simulink model "SDOF_v1"  (R2026a)
settings: Solver=VariableStepAuto  StopTime=200
InitFcn:
  | model_path = fileparts(get_param(bdroot, 'FileName'));
  | parent_path = fileparts(model_path);
  | run(fullfile(parent_path, 'scripts', 'InitFcn.m'));
undefined symbols (not defined in the file): data, envP
libraries: simulink x2
settings Model: Creator=awint  LastModifiedBy=benjaminbrobst

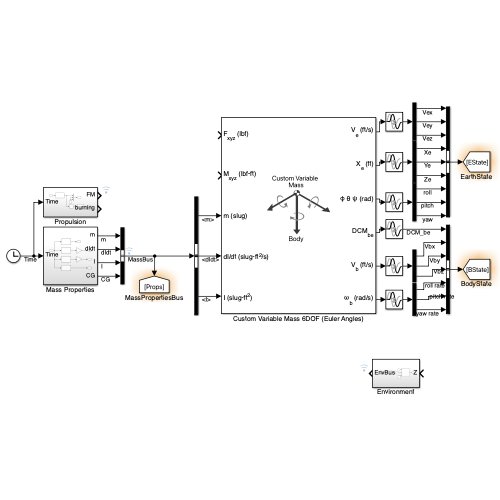
[thumbnail: Simulink's stored preview of the top-level diagram]
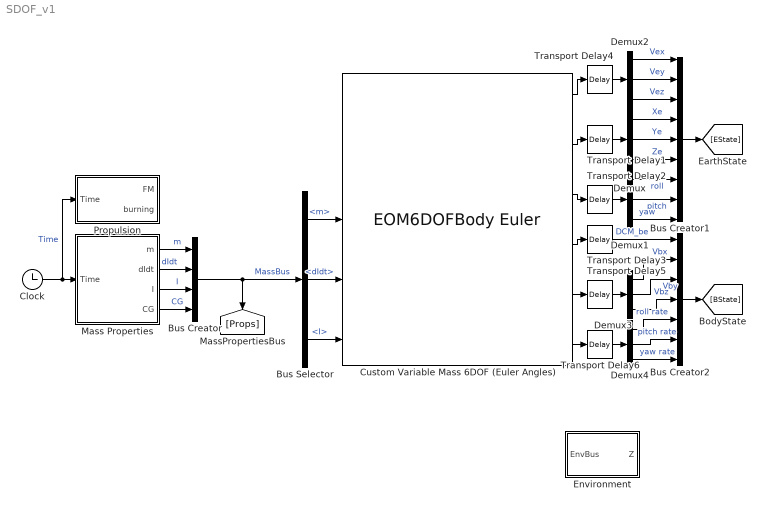
== system SDOF_v1 ==
  Bus Creator : BusCreator  Inputs=4
  Bus Creator1 : BusCreator  Inputs=9
  Bus Creator2 : BusCreator  Inputs=7
  Bus Selector : BusSelector  OutputSignals=m,dIdt,I
  Clock : Clock
  Custom Variable Mass 6DOF (Euler Angles) : EOM6DOFBodyEuler  units=English (velocity in ft/s)  mtype=Custom Variable
  Demux{,1..4} (5 alike) : Demux  Outputs=3
  Environment : Subsystem
  Mass Properties : Subsystem
  Propulsion : Subsystem
  Transport Delay{1..6} (6 alike) : TransportDelay  DelayTime=0.001
  wires:
  Clock/1 -> Propulsion/1(Time), Mass Properties/1(Time)  "Time"
  Custom Variable Mass 6DOF (Euler Angles)/1 -> Transport Delay4/1
  Custom Variable Mass 6DOF (Euler Angles)/2 -> Transport Delay1/1
  Custom Variable Mass 6DOF (Euler Angles)/3 -> Transport Delay2/1
  Custom Variable Mass 6DOF (Euler Angles)/4 -> Transport Delay3/1
  Custom Variable Mass 6DOF (Euler Angles)/5 -> Transport Delay5/1
  Custom Variable Mass 6DOF (Euler Angles)/6 -> Transport Delay6/1
  Mass Properties/4(CG) -> Bus Creator/4  "CG"
  Mass Properties/3(I) -> Bus Creator/3  "I"
  Mass Properties/2(dIdt) -> Bus Creator/2  "dIdt"
  Mass Properties/1(m) -> Bus Creator/1  "m"
  Bus Creator/1 -> Bus Selector/1, [Props]  "MassBus"
  Bus Selector/1 -> Custom Variable Mass 6DOF (Euler Angles)/3  "<m>"
  Bus Selector/2 -> Custom Variable Mass 6DOF (Euler Angles)/4  "<dIdt>"
  Bus Selector/3 -> Custom Variable Mass 6DOF (Euler Angles)/5  "<I>"
  Transport Delay4/1 -> Demux2/1
  Transport Delay1/1 -> Demux/1
  Transport Delay2/1 -> Demux1/1
  Transport Delay5/1 -> Demux3/1
  Transport Delay6/1 -> Demux4/1
  Demux2/1 -> Bus Creator1/1  "Vex"
  Demux2/2 -> Bus Creator1/2  "Vey"
  Demux2/3 -> Bus Creator1/3  "Vez"
  Demux/1 -> Bus Creator1/4  "Xe"
  Demux/2 -> Bus Creator1/5  "Ye"
  Demux/3 -> Bus Creator1/6  "Ze"
  Demux1/1 -> Bus Creator1/7  "roll"
  Demux1/2 -> Bus Creator1/8  "pitch"
  Demux1/3 -> Bus Creator1/9  "yaw"
  Demux4/3 -> Bus Creator2/7  "yaw rate"
  Demux4/2 -> Bus Creator2/6  "pitch rate"
  Demux4/1 -> Bus Creator2/5  "roll rate"
  Demux3/3 -> Bus Creator2/4  "Vbz"
  Demux3/2 -> Bus Creator2/3  "Vby"
  Demux3/1 -> Bus Creator2/2  "Vbx"
  Transport Delay3/1 -> Bus Creator2/1  "DCM_be"
  Bus Creator1/1 -> [EState]
  Bus Creator2/1 -> [BState]

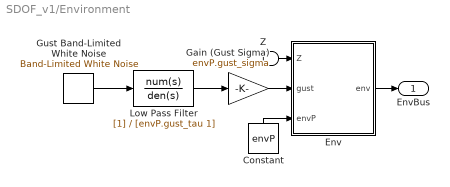
== system SDOF_v1/Environment ==
  Z : Inport
  Constant : Constant  Value=envP  OutDataTypeStr=Bus: slBus2
  Env : MATLAB Function  TreatAsAtomicUnit=on
  Gain (Gust Sigma) : Gain  Gain=envP.gust_sigma
  Gust Band-Limited White Noise : simulink/Sources/Band-Limited White Noise  Cov=1  Ts=0.1  seed=envP.gust_seed
  Low Pass Filter : TransferFcn  Denominator=[envP.gust_tau 1]
  EnvBus : Outport  OutDataTypeStr=Bus: EnvBus
  wires:
  Env/1(env) -> EnvBus/1
  Z/1 -> Env/1(Z)
  Gain (Gust Sigma)/1 -> Env/2(gust)
  Constant/1 -> Env/3(envP)
  Gust Band-Limited White Noise/1 -> Low Pass Filter/1
  Low Pass Filter/1 -> Gain (Gust Sigma)/1

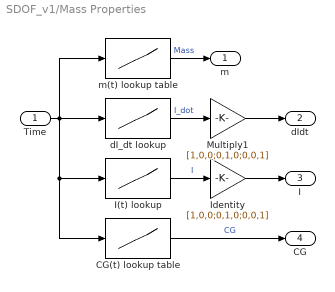
== system SDOF_v1/Mass Properties ==
  Time : Inport
  CG(t) lookup table : Lookup_n-D  NumberOfTableDimensions=1  BreakpointsForDimension1=data.time_vec  Table=data.CG_vec  ExtrapMethod=Clip  UseLastTableValue=on  InternalRulePriority=Speed  RndMeth=Simplest
  I(t) lookup : Lookup_n-D  NumberOfTableDimensions=1  BreakpointsForDimension1=data.time_vec  Table=data.I_vec  ExtrapMethod=Clip  UseLastTableValue=on  InternalRulePriority=Speed  RndMeth=Simplest
  Identity : Gain  Gain=[1,0,0;0,1,0;0,0,1]
  Multiply1 : Gain  Gain=[1,0,0;0,1,0;0,0,1]
  dI_dt lookup : Lookup_n-D  NumberOfTableDimensions=1  BreakpointsForDimension1=data.time_vec(1:end-1)  Table=data.dI_dt_vec  ExtrapMethod=Clip  UseLastTableValue=on  InternalRulePriority=Speed  RndMeth=Simplest
  m(t) lookup table : Lookup_n-D  NumberOfTableDimensions=1  BreakpointsForDimension1=data.time_vec  Table=data.tot_mass_vec  ExtrapMethod=Clip  UseLastTableValue=on  InternalRulePriority=Speed  RndMeth=Simplest
  m : Outport
  dIdt : Outport  Port=2
  I : Outport  Port=3
  CG : Outport  Port=4
  wires:
  Time/1 -> CG(t) lookup table/1, I(t) lookup/1, dI_dt lookup/1, m(t) lookup table/1
  m(t) lookup table/1 -> m/1  "Mass"
  I(t) lookup/1 -> Identity/1  "I"
  Identity/1 -> I/1
  CG(t) lookup table/1 -> CG/1  "CG"
  dI_dt lookup/1 -> Multiply1/1  "I_dot"
  Multiply1/1 -> dIdt/1

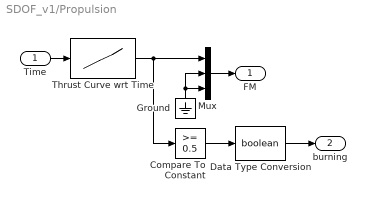
== system SDOF_v1/Propulsion ==
  Time : Inport
  Compare To Constant : simulink/Logic and Bit Operations/Compare To Constant  relop=>=  const=0.5  OutDataTypeStr=boolean
  Data Type Conversion : DataTypeConversion  OutDataTypeStr=boolean  SaturateOnIntegerOverflow=off  RndMeth=Floor
  Ground : Ground
  Mux : Mux  Inputs=3
  Thrust Curve wrt Time : Lookup_n-D  NumberOfTableDimensions=1  BreakpointsForDimension1=data.time_vec  Table=data.thrust_vec  ExtrapMethod=Clip  UseLastTableValue=on  InternalRulePriority=Speed  RndMeth=Simplest
  FM : Outport
  burning : Outport  Port=2
  wires:
  Time/1 -> Thrust Curve wrt Time/1
  Mux/1 -> FM/1
  Ground/1 -> Mux/3, Mux/2
  Thrust Curve wrt Time/1 -> Compare To Constant/1, Mux/1
  Compare To Constant/1 -> Data Type Conversion/1
  Data Type Conversion/1 -> burning/1

== matlab function SDOF_v1/Environment/Env ==
  data: Z input; env output Bus: EnvBus; gust input; envP input
function env = Environment_blk(Z, gust,envP)
% Edit the function Environment.m in MATLAB proper for easier commits.
env = Environment(Z,gust,envP);
end
